simulink model "lab1primer"  (R2012b)
settings: Solver=ode45  StartTime=0.0  StopTime=50  RelTol=1e-3
undefined symbols (not defined in the file): des, gcbh
settings Model: Creator=Student  LastModifiedBy=Student

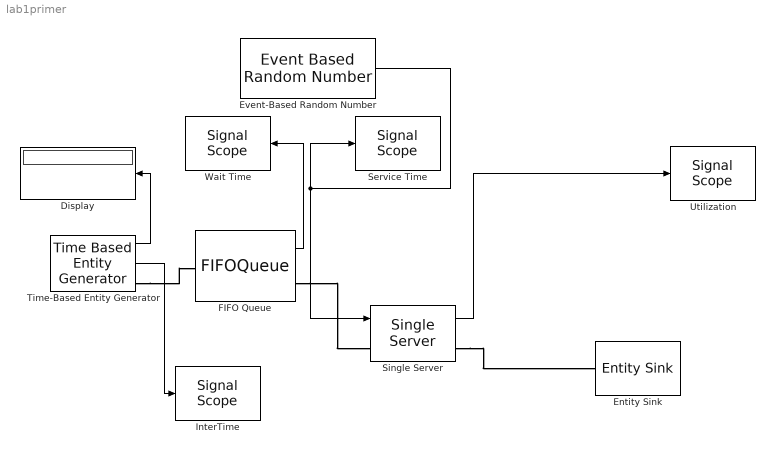
== system lab1primer ==
  Display : Display
  Entity Sink : EntitySink
  Event-Based Random Number : EventBasedRandomNumber  Distribution=Uniform  meanExp=1.5  minUnif=1.5  maxUnif=2.5
  FIFO Queue : FIFOQueue  StatAverageWait=on
      settings: OutputPortMap=o2
  InterTime : SignalScope  LoadFcn=des.scope.CallbackSupport('seLoadFcn',gcbh)  StartFcn=des.scope.CallbackSupport('seStartFcn',gcbh)  StopFcn=des.scope.CallbackSupport('seStopFcn',gcbh)
      settings: CopyFcn=des.scope.CallbackSupport('seCopyFcn',gcbh)  DeleteFcn=des.scope.CallbackSupport('seDeleteFcn',gcbh)  PreSaveFcn=des.scope.CallbackSupport('sePreSaveFcn',gcbh)  NameChangeFcn=des.scope.CallbackSupport('seNameChangeFcn',gcbh)  OpenFcn=des.scope.CallbackSupport('seOpenFcn',gcbh)
  Service Time : SignalScope  LoadFcn=des.scope.CallbackSupport('seLoadFcn',gcbh)  StartFcn=des.scope.CallbackSupport('seStartFcn',gcbh)  StopFcn=des.scope.CallbackSupport('seStopFcn',gcbh)
      settings: CopyFcn=des.scope.CallbackSupport('seCopyFcn',gcbh)  DeleteFcn=des.scope.CallbackSupport('seDeleteFcn',gcbh)  PreSaveFcn=des.scope.CallbackSupport('sePreSaveFcn',gcbh)  NameChangeFcn=des.scope.CallbackSupport('seNameChangeFcn',gcbh)  OpenFcn=des.scope.CallbackSupport('seOpenFcn',gcbh)
  Single Server : SingleServer  ServiceTimeFrom=Signal port t  StatUtilization=on
      settings: OutputPortMap=o5
  Time-Based Entity Generator : TimeBasedEntityGenerator  Period=2  StatNumberDeparted=on  StatAverageIntergenerationTime=on
      settings: OutputPortMap=o0,o2
  Utilization : SignalScope  LoadFcn=des.scope.CallbackSupport('seLoadFcn',gcbh)  StartFcn=des.scope.CallbackSupport('seStartFcn',gcbh)  StopFcn=des.scope.CallbackSupport('seStopFcn',gcbh)
      settings: CopyFcn=des.scope.CallbackSupport('seCopyFcn',gcbh)  DeleteFcn=des.scope.CallbackSupport('seDeleteFcn',gcbh)  PreSaveFcn=des.scope.CallbackSupport('sePreSaveFcn',gcbh)  NameChangeFcn=des.scope.CallbackSupport('seNameChangeFcn',gcbh)  OpenFcn=des.scope.CallbackSupport('seOpenFcn',gcbh)
  Wait Time : SignalScope  LoadFcn=des.scope.CallbackSupport('seLoadFcn',gcbh)  StartFcn=des.scope.CallbackSupport('seStartFcn',gcbh)  StopFcn=des.scope.CallbackSupport('seStopFcn',gcbh)
      settings: CopyFcn=des.scope.CallbackSupport('seCopyFcn',gcbh)  DeleteFcn=des.scope.CallbackSupport('seDeleteFcn',gcbh)  PreSaveFcn=des.scope.CallbackSupport('sePreSaveFcn',gcbh)  NameChangeFcn=des.scope.CallbackSupport('seNameChangeFcn',gcbh)  OpenFcn=des.scope.CallbackSupport('seOpenFcn',gcbh)
  wires:
  Single Server/1 -> Utilization/1
  Event-Based Random Number/1 -> Single Server/1, Service Time/1
  Time-Based Entity Generator/1 -> Display/1
  Time-Based Entity Generator/2 -> InterTime/1
  FIFO Queue/1 -> Wait Time/1
  connections:
  Single Server/RConn1 -- Entity Sink/LConn1
  FIFO Queue/RConn1 -- Single Server/LConn1
  Time-Based Entity Generator/RConn1 -- FIFO Queue/LConn1
